simulink model "BLDC_2024b"  (R2024b)
settings: Solver=VariableStepAuto  StartTime=0.0  StopTime=10.0  RelTol=1e-3
libraries: spsMosfetLib x6, simulink x6, spsControlledVoltageSourceLib x1, slpidlib x1, spsPermanentMagnetSynchronousMachineLib x1, sps_lib x1
settings Model: Creator=Test  LastModifiedBy=Test

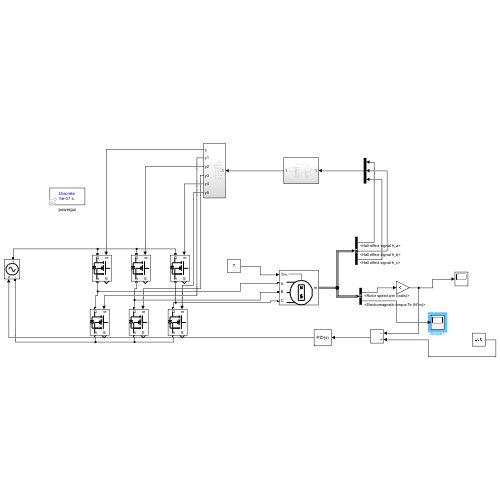
[thumbnail: Simulink's stored preview of the top-level diagram]
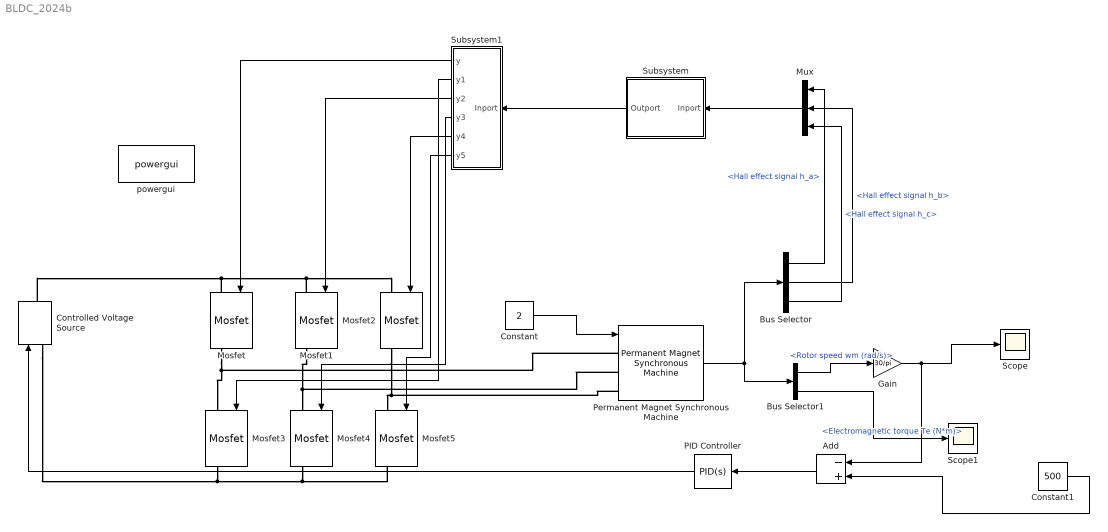
== system BLDC_2024b ==
  Add : Sum  Inputs=-+
  Bus Selector : BusSelector  OutputSignals=Hall effect signal h_a,Hall effect signal h_b,Hall effect signal h_c
  Bus Selector1 : BusSelector  OutputSignals=Rotor speed wm (rad/s),Electromagnetic torque Te (N*m)
  Constant : Constant  Value=2
  Constant1 : Constant  Value=500
  Controlled Voltage Source : spsControlledVoltageSourceLib/Controlled Voltage Source  Initialize=on  Source_Type=DC  Amplitude=0  Phase=0  Frequency=0  Measurements=None
  Gain : Gain  Gain=30/pi
  Mosfet{,1..5} (6 alike) : spsMosfetLib/Mosfet  Ron=0.1  Lon=0  Rd=0.01  Vfd=0  IC=0  Rs=1e5  Cs=inf  Measurements=on
  Mux : Mux  Inputs=3
  PID Controller : slpidlib/PID Controller  Controller=PID  Form=Parallel  TimeDomain=Continuous-time  UseExternalTs=off  SampleTime=-1  IntegratorMethod=Forward Euler  FilterMethod=Forward Euler  ControllerParametersSource=internal  P=0.01  I=12.777  UseKiTs=off  D=12.53  UseExternalDerivativeSource=off  N=0  UseFilter=on  TunerSelectOption=Transfer Function Based (PID Tuner App)  InitialConditionSource=internal  InitialConditionForIntegrator=0  InitialConditionForFilter=0  DifferentiatorICPrevScaledInput=0  ExternalReset=none  TrackingMode=off  Kt=1  LimitOutput=off  SatLimitsSource=internal  UpperSaturationLimit=inf  LowerSaturationLimit=-inf  LinearizeAsGain=on  AntiWindupMode=none  Kb=1  LimitIntegrator=off  UpperIntegratorSaturationLimit=inf  LowerIntegratorSaturationLimit=-inf  POutMin=[]  POutMax=[]  IOutMin=[]  IOutMax=[]  DOutMin=[]  DOutMax=[]  NOutMin=[]  NOutMax=[]  SumOutMin=[]  SumOutMax=[]  SaturationOutMin=[]  SaturationOutMax=[]  PParamMin=[]  PParamMax=[]  IParamMin=[]  IParamMax=[]  DParamMin=[]  DParamMax=[]  NParamMin=[]  NParamMax=[]  KbParamMin=[]  KbParamMax=[]  KtParamMin=[]  KtParamMax=[]  KbOutMin=[]  KbOutMax=[]  KtOutMin=[]  KtOutMax=[]  IntegratorOutMin=[]  IntegratorOutMax=[]  FilterOutMin=[]  FilterOutMax=[]  SumI1OutMin=[]  SumI1OutMax=[]  SumI2OutMin=[]  SumI2OutMax=[]  SumI3OutMin=[]  SumI3OutMax=[]  SumI4OutMin=[]  SumI4OutMax=[]  SumDOutMin=[]  SumDOutMax=[]  DifferentiatorOutMin=[]  DifferentiatorOutMax=[]  FilterDiffOutCoefMin=[]  FilterDiffOutCoefMax=[]  ReciprocalOutMin=[]  ReciprocalOutMax=[]  SumDenOutMin=[]  SumDenOutMax=[]  SumNumOutMin=[]  SumNumOutMax=[]  DivideOutMin=[]  DivideOutMax=[]  UdiffTsProdOutMin=[]  UdiffTsProdOutMax=[]  NTsProdOutMin=[]  NTsProdOutMax=[]  UintegralTsProdOutMin=[]  UintegralTsProdOutMax=[]  UngainTsProdOutMin=[]  UngainTsProdOutMax=[]  ClampingZeroOutDataTypeStr=Inherit: Inherit via back propagation  ClampingZeroOutMin=[]  ClampingZeroOutMax=[]  FilterDenConstantOutDataTypeStr=Inherit: Inherit via back propagation  FilterDenConstantOutMin=[]  FilterDenConstantOutMax=[]  PCopyOutDataTypeStr=Inherit: Inherit via back propagation  PCopyOutMin=[]  PCopyOutMax=[]  NCopyOutDataTypeStr=Inherit: Inherit via back propagation  NCopyOutMin=[]  NCopyOutMax=[]  IntegratorContinuousStateAttributes=''  IntegratorStateMustResolveToSignalObject=off  IntegratorRTWStateStorageClass=Auto  FilterContinuousStateAttributes=''  FilterStateMustResolveToSignalObject=off  FilterRTWStateStorageClass=Auto  ParallelPVariant=InternalParameters  IdealPVariant=Disabled  IVariant=InternalParameters  DVariant=InternalParameters  IntegratorVariant=Continuous  SatVariant=Disabled  AWVariant=Passthrough  PCopyVariant=Disabled  TRVariant=Disabled  FdbkBlocksVariant=Forward  IdealPFdbkVariant=Disabled  SatFdbkVariant=Disabled  DerivativeFilterVariant=ContFilter  NVariant=InternalParameters  NCopyVariant=Disabled  FilterICVariant=InternalICsFilter  IntegratorICVariant=InternalICs  ExternalResetVariant=Disabled  TRSumVariant=Passthrough  SumFdbkVariant=Disabled  SumVariant=Sum_PID  TsampFilterVariant=InternalTs  TsampNgainVariant=Passthrough  TsampIntegralVariant=Disabled_SignalSpec  ExternalSaturationOutDataTypeStr=Inherit: Same as second input  DerivativeSourceVariant=ErrorSignal  PreIntVariant=InternalPreInt
  Permanent Magnet Synchronous Machine : spsPermanentMagnetSynchronousMachineLib/Permanent Magnet Synchronous Machine  NbPhases=3  FluxDistribution=Trapezoidal  RotorType=Round  MechanicalLoad=Torque Tm  PresetModel=No  ShowDetailedParameters=on  MeasurementBus=off  Resistance=0.7  Inductance=2.7e-3  dqInductances=[8.5e-3,8.5e-3]  La=0.000395  MachineConstant=Flux linkage established by magnets (V.s)  Flux=0.1194  VoltageCst=100.0283  TorqueCst=0.9552  Flat=120  Mechanical=[0.0027 0.0004924 4 0]  PolePairs=4  InitialConditions=[0,0, 0,0]  InitialConditions5ph=[0 0 0 0 0 0]  RefAngle=90 degrees behind phase A axis (modified Park)  IterativeDiscreteModel=Trapezoidal non iterative  TsBlock=-1  TsPowergui=0
  Scope : Scope
  Scope1 : Scope
  Subsystem : Subsystem
  Subsystem1 : Subsystem
  powergui : sps_lib/powergui  Priority=1  SimulationMode=Discrete  SampleTime=5e-7  frequency=60  Iterations=50  frequencyindice=0  Pbase=100e6  ErrMax=1e-4  UnitsV=kV  UnitsW=MW  buscounter=0  FunctionMessages=off  echomessages=off  EnableUseOfTLC=off  CurrentSourceSwitches=off  DisableSnubberDevices=off  DisableRonSwitches=off  DisableVfSwitches=off  DisplayEquations=off  AutomaticDiscreteSolvers=off  SolverType=Tustin/Backward Euler (TBE)  Interpol=off  ExternalGateDelay=off  methode=off  Ts=100  x0status=blocks  SPID=on  SwTol=0  HookPort=off  NonlinearTolerance=1e-4  nMaxIteration=100  ContinueOnMaxIteration=off  RestoreLinks=warning  ResistiveCurrentMeasurement=off  Frange=[0:2:500]  Ylog=off  Xlog=on  ShowGrid=off  save=off  variable=ZData  structure=0  ZoomFFT=off  StartTime=0.0  cycles=1  DisplayStyle=1  fundamental=60  FreqAxis=off  MaxFrequency=1000  frequencyindicesteady=1  RmsSteady=1  display=off
  wires:
  Subsystem/1(Outport) -> Subsystem1/1(Inport)
  Subsystem1/1(y) -> Mosfet/1
  Subsystem1/2(y1) -> Mosfet3/1
  Subsystem1/3(y2) -> Mosfet1/1
  Subsystem1/4(y3) -> Mosfet4/1
  Subsystem1/5(y4) -> Mosfet2/1
  Subsystem1/6(y5) -> Mosfet5/1
  Constant/1 -> Permanent Magnet Synchronous Machine/1
  Permanent Magnet Synchronous Machine/1 -> Bus Selector/1, Bus Selector1/1
  Gain/1 -> Add/1, Scope/1
  Bus Selector1/1 -> Gain/1  "<Rotor speed wm (rad/s)>"
  Bus Selector1/2 -> Scope1/1  "<Electromagnetic torque Te (N*m)>"
  Constant1/1 -> Add/2
  Mux/1 -> Subsystem/1(Inport)
  Bus Selector/1 -> Mux/1  "<Hall effect signal h_a>"
  Bus Selector/2 -> Mux/2  "<Hall effect signal h_b>"
  Bus Selector/3 -> Mux/3  "<Hall effect signal h_c>"
  Add/1 -> PID Controller/1
  PID Controller/1 -> Controlled Voltage Source/1
  connections:
  Controlled Voltage Source/RConn1 -- Mosfet/LConn1 -- Mosfet1/LConn1 -- Mosfet2/LConn1
  Controlled Voltage Source/LConn1 -- Mosfet3/RConn1 -- Mosfet4/RConn1 -- Mosfet5/RConn1
  Mosfet/RConn1 -- Permanent Magnet Synchronous Machine/LConn1 -- Mosfet3/LConn1
  Mosfet1/RConn1 -- Permanent Magnet Synchronous Machine/LConn2 -- Mosfet4/LConn1
  Mosfet2/RConn1 -- Permanent Magnet Synchronous Machine/LConn3 -- Mosfet5/LConn1

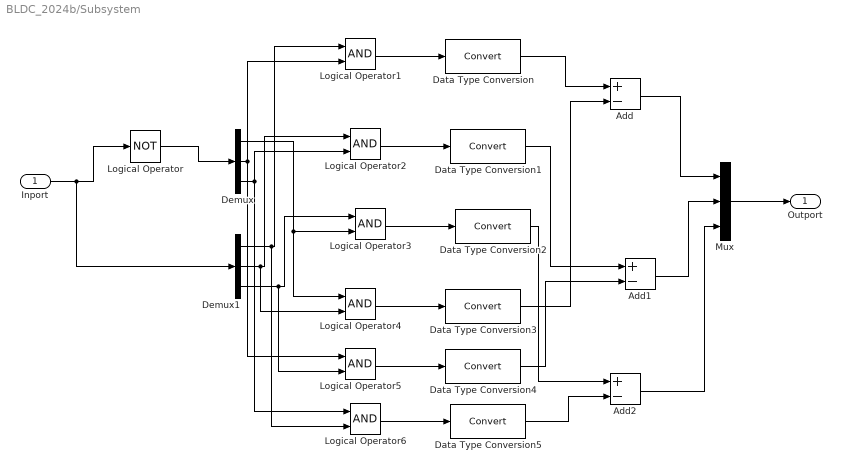
== system BLDC_2024b/Subsystem ==
  Inport : Inport
  Add : Sum  Inputs=+-
  Add1 : Sum  Inputs=+-
  Add2 : Sum  Inputs=+-
  Data Type Conversion{,1..5} (6 alike) : DataTypeConversion  SaturateOnIntegerOverflow=off  RndMeth=Floor
  Demux : Demux  Outputs=3
  Demux1 : Demux  Outputs=3
  Logical Operator : Logic  Operator=NOT  AllPortsSameDT=off  OutDataTypeStr=boolean
  Logical Operator{1..6} (6 alike) : Logic  AllPortsSameDT=off  OutDataTypeStr=boolean
  Mux : Mux  Inputs=3
  Outport : Outport
  wires:
  Data Type Conversion3/1 -> Add/2
  Demux/3 -> Logical Operator6/1, Logical Operator2/2
  Logical Operator2/1 -> Data Type Conversion1/1
  Demux1/1 -> Logical Operator6/2, Logical Operator1/1
  Logical Operator/1 -> Demux/1
  Mux/1 -> Outport/1
  Demux/2 -> Logical Operator5/1, Logical Operator1/2
  Demux1/3 -> Logical Operator5/2, Logical Operator3/1
  Demux/1 -> Logical Operator3/2, Logical Operator4/1
  Data Type Conversion5/1 -> Add2/2
  Add1/1 -> Mux/2
  Logical Operator6/1 -> Data Type Conversion5/1
  Logical Operator3/1 -> Data Type Conversion2/1
  Logical Operator4/1 -> Data Type Conversion3/1
  Data Type Conversion/1 -> Add/1
  Inport/1 -> Demux1/1, Logical Operator/1
  Data Type Conversion2/1 -> Add2/1
  Data Type Conversion4/1 -> Add1/2
  Demux1/2 -> Logical Operator4/2, Logical Operator2/1
  Add/1 -> Mux/1
  Add2/1 -> Mux/3
  Logical Operator1/1 -> Data Type Conversion/1
  Logical Operator5/1 -> Data Type Conversion4/1
  Data Type Conversion1/1 -> Add1/1

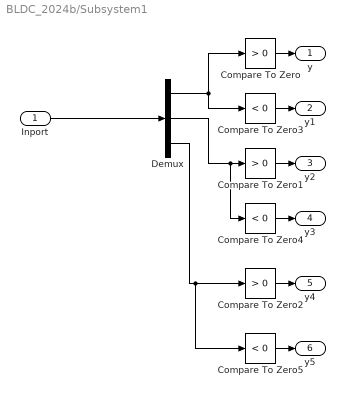
== system BLDC_2024b/Subsystem1 ==
  Inport : Inport
  Compare To Zero : simulink/Logic and Bit Operations/Compare To Zero  relop=>  OutDataTypeStr=boolean
  Compare To Zero1 : simulink/Logic and Bit Operations/Compare To Zero  relop=>  OutDataTypeStr=boolean
  Compare To Zero2 : simulink/Logic and Bit Operations/Compare To Zero  relop=>  OutDataTypeStr=boolean
  Compare To Zero3 : simulink/Logic and Bit Operations/Compare To Zero  relop=<  OutDataTypeStr=boolean
  Compare To Zero4 : simulink/Logic and Bit Operations/Compare To Zero  relop=<  OutDataTypeStr=boolean
  Compare To Zero5 : simulink/Logic and Bit Operations/Compare To Zero  relop=<  OutDataTypeStr=boolean
  Demux : Demux  Outputs=3
  y : Outport
  y1 : Outport  Port=2
  y2 : Outport  Port=3
  y3 : Outport  Port=4
  y4 : Outport  Port=5
  y5 : Outport  Port=6
  wires:
  Demux/1 -> Compare To Zero/1, Compare To Zero3/1
  Inport/1 -> Demux/1
  Demux/3 -> Compare To Zero5/1, Compare To Zero2/1
  Demux/2 -> Compare To Zero4/1, Compare To Zero1/1
  Compare To Zero1/1 -> y2/1
  Compare To Zero2/1 -> y4/1
  Compare To Zero5/1 -> y5/1
  Compare To Zero3/1 -> y1/1
  Compare To Zero4/1 -> y3/1
  Compare To Zero/1 -> y/1
